simulink model "Trigger_Test"  (R2022b)
settings: Solver=VariableStepAuto  StartTime=0.0  StopTime=10.0  RelTol=1e-3
settings Model: Creator=CSMotor  LastModifiedBy=CSMotor

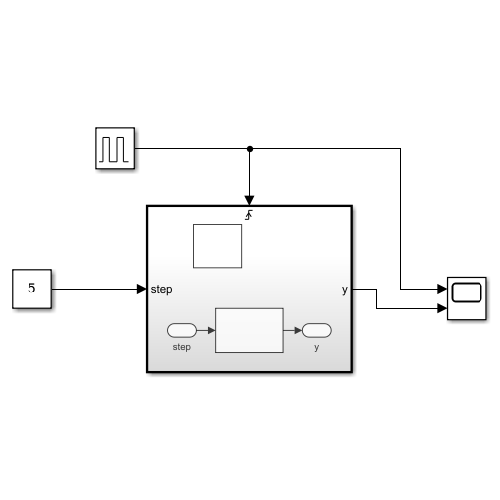
[thumbnail: Simulink's stored preview of the top-level diagram]
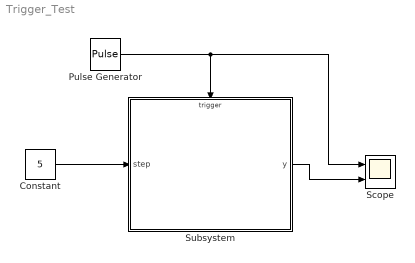
== system Trigger_Test ==
  Constant : Constant  Value=5
  Pulse Generator : DiscretePulseGenerator  PulseType=Time based  Period=1  PulseWidth=5
  Scope : Scope  NumInputPorts=2
  Subsystem : Subsystem
  wires:
  Pulse Generator/1 -> Scope/1, Subsystem/Trigger
  Constant/1 -> Subsystem/1(step)
  Subsystem/1(y) -> Scope/2

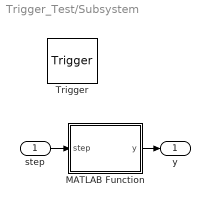
== system Trigger_Test/Subsystem ==
  step : Inport
  Trigger : TriggerPort  VariantControl=(inherit)  PortDimensions=1
  MATLAB Function : MATLAB Function  TreatAsAtomicUnit=on
  y : Outport
  wires:
  step/1 -> MATLAB Function/1(step)
  MATLAB Function/1(y) -> y/1

== matlab function Trigger_Test/Subsystem/MATLAB Function ==
  data: step input; y output
function y = fcn(step)
%#codegen
persistent acc
if isempty(acc)
    acc = 0;
end
acc = acc + step;
y = acc;
